simulink library "Inverter"  (R2026a)
settings: Solver=VariableStepAuto
undefined symbols (not defined in the file): inverterCfg
settings Model: Creator=24322  LastModifiedBy=24322

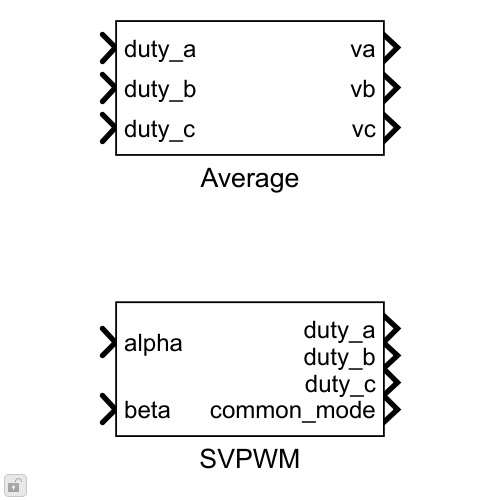
[thumbnail: Simulink's stored preview of the top-level diagram]
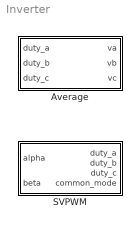
== system Inverter ==
  Average : Subsystem
  SVPWM : Subsystem

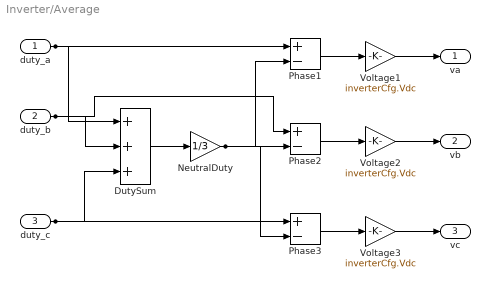
== system Inverter/Average ==
  duty_a : Inport
  duty_b : Inport  Port=2
  duty_c : Inport  Port=3
  DutySum : Sum  Inputs=+++
  NeutralDuty : Gain  Gain=1/3
  Phase1 : Sum  Inputs=+-
  Phase2 : Sum  Inputs=+-
  Phase3 : Sum  Inputs=+-
  Voltage1 : Gain  Gain=inverterCfg.Vdc
  Voltage2 : Gain  Gain=inverterCfg.Vdc
  Voltage3 : Gain  Gain=inverterCfg.Vdc
  va : Outport
  vb : Outport  Port=2
  vc : Outport  Port=3
  wires:
  Voltage3/1 -> vc/1
  Phase3/1 -> Voltage3/1
  duty_c/1 -> DutySum/3, Phase3/1
  Voltage2/1 -> vb/1
  Phase2/1 -> Voltage2/1
  duty_b/1 -> Phase2/1, DutySum/2
  Voltage1/1 -> va/1
  Phase1/1 -> Voltage1/1
  NeutralDuty/1 -> Phase1/2, Phase2/2, Phase3/2
  duty_a/1 -> DutySum/1, Phase1/1
  DutySum/1 -> NeutralDuty/1

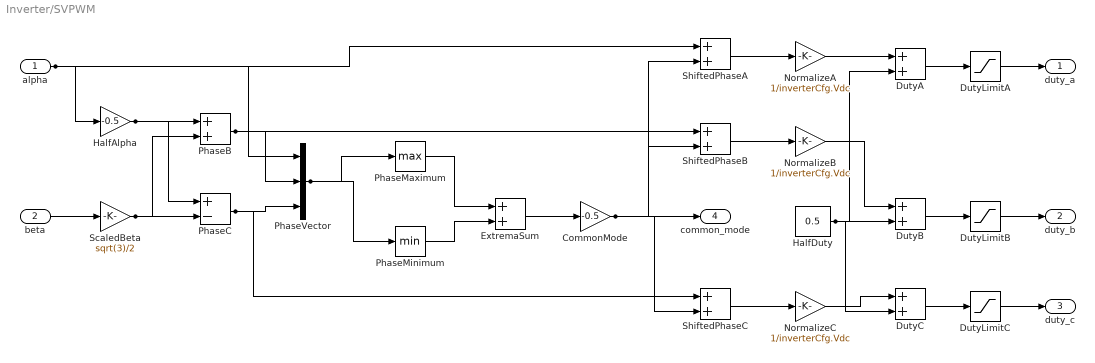
== system Inverter/SVPWM ==
  alpha : Inport
  beta : Inport  Port=2
  CommonMode : Gain  Gain=-0.5
  DutyA : Sum
  DutyB : Sum
  DutyC : Sum
  DutyLimitA : Saturate  UpperLimit=1-inverterCfg.MinDuty  LowerLimit=inverterCfg.MinDuty
  DutyLimitB : Saturate  UpperLimit=1-inverterCfg.MinDuty  LowerLimit=inverterCfg.MinDuty
  DutyLimitC : Saturate  UpperLimit=1-inverterCfg.MinDuty  LowerLimit=inverterCfg.MinDuty
  ExtremaSum : Sum
  HalfAlpha : Gain  Gain=-0.5
  HalfDuty : Constant  Value=0.5
  NormalizeA : Gain  Gain=1/inverterCfg.Vdc
  NormalizeB : Gain  Gain=1/inverterCfg.Vdc
  NormalizeC : Gain  Gain=1/inverterCfg.Vdc
  PhaseB : Sum
  PhaseC : Sum  Inputs=+-
  PhaseMaximum : MinMax  Function=max
  PhaseMinimum : MinMax
  PhaseVector : Mux  Inputs=3
  ScaledBeta : Gain  Gain=sqrt(3)/2
  ShiftedPhaseA : Sum
  ShiftedPhaseB : Sum
  ShiftedPhaseC : Sum
  duty_a : Outport
  duty_b : Outport  Port=2
  duty_c : Outport  Port=3
  common_mode : Outport  Port=4
  wires:
  PhaseC/1 -> PhaseVector/3, ShiftedPhaseC/1
  PhaseB/1 -> ShiftedPhaseB/1, PhaseVector/2
  alpha/1 -> HalfAlpha/1, ShiftedPhaseA/1, PhaseVector/1
  beta/1 -> ScaledBeta/1
  PhaseVector/1 -> PhaseMinimum/1, PhaseMaximum/1
  PhaseMaximum/1 -> ExtremaSum/1
  PhaseMinimum/1 -> ExtremaSum/2
  ExtremaSum/1 -> CommonMode/1
  CommonMode/1 -> common_mode/1, ShiftedPhaseA/2, ShiftedPhaseB/2, ShiftedPhaseC/2
  ShiftedPhaseA/1 -> NormalizeA/1
  NormalizeA/1 -> DutyA/1
  HalfDuty/1 -> DutyB/2, DutyC/2, DutyA/2
  DutyA/1 -> DutyLimitA/1
  DutyLimitA/1 -> duty_a/1
  ShiftedPhaseB/1 -> NormalizeB/1
  NormalizeB/1 -> DutyB/1
  DutyB/1 -> DutyLimitB/1
  DutyLimitB/1 -> duty_b/1
  ShiftedPhaseC/1 -> NormalizeC/1
  NormalizeC/1 -> DutyC/1
  DutyC/1 -> DutyLimitC/1
  DutyLimitC/1 -> duty_c/1
  HalfAlpha/1 -> PhaseB/1, PhaseC/1
  ScaledBeta/1 -> PhaseB/2, PhaseC/2
